simulink model "PID_SCHEME"  (R2024b)
settings: Solver=VariableStepAuto  StartTime=0.0  StopTime=10.0  RelTol=1e-3
undefined symbols (not defined in the file): a, b
libraries: slpidlib x1, px4Sensorslib x1, px4Peripheralslib x1
settings Model: Creator=xippa  LastModifiedBy=xippa

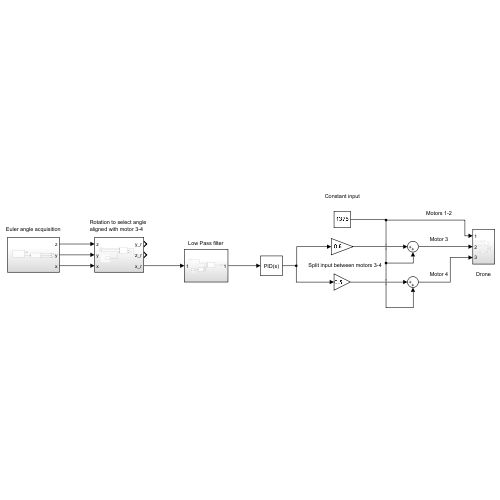
[thumbnail: Simulink's stored preview of the top-level diagram]
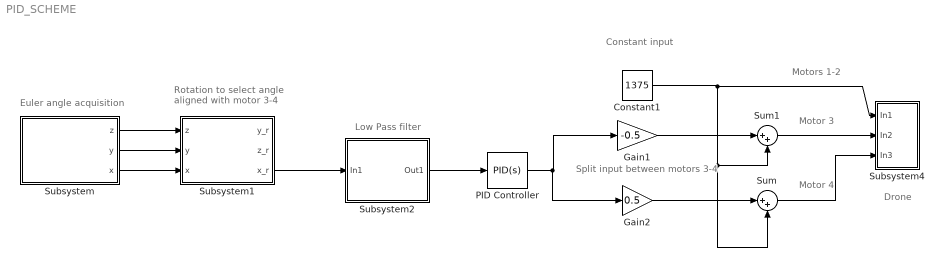
== system PID_SCHEME ==
  note: Drone
  note: Motor 4
  note: Motor 3
  note: Motors 1-2
  note: Constant input
  note: Split input between motors 3-4
  note: Low Pass filter
  note: Rotation to select angle
      | aligned with motor 3-4
  note: Euler angle acquisition
  Constant1 : Constant  Value=1375  SampleTime=0.001
  Gain1 : Gain  Gain=-0.5
  Gain2 : Gain  Gain=0.5
  PID Controller : slpidlib/PID Controller  Controller=PID  Form=Parallel  TimeDomain=Continuous-time  UseExternalTs=off  SampleTime=-1  IntegratorMethod=Forward Euler  FilterMethod=Forward Euler  ControllerParametersSource=internal  P=450  I=250  UseKiTs=off  D=100  UseExternalDerivativeSource=off  N=100  UseFilter=on  TunerSelectOption=Transfer Function Based (PID Tuner App)  InitialConditionSource=internal  InitialConditionForIntegrator=0  InitialConditionForFilter=0  DifferentiatorICPrevScaledInput=0  ExternalReset=none  TrackingMode=off  Kt=1  LimitOutput=off  SatLimitsSource=internal  UpperSaturationLimit=inf  LowerSaturationLimit=-inf  LinearizeAsGain=on  AntiWindupMode=none  Kb=1  LimitIntegrator=off  UpperIntegratorSaturationLimit=inf  LowerIntegratorSaturationLimit=-inf  POutMin=[]  POutMax=[]  IOutMin=[]  IOutMax=[]  DOutMin=[]  DOutMax=[]  NOutMin=[]  NOutMax=[]  SumOutMin=[]  SumOutMax=[]  SaturationOutMin=[]  SaturationOutMax=[]  PParamMin=[]  PParamMax=[]  IParamMin=[]  IParamMax=[]  DParamMin=[]  DParamMax=[]  NParamMin=[]  NParamMax=[]  KbParamMin=[]  KbParamMax=[]  KtParamMin=[]  KtParamMax=[]  KbOutMin=[]  KbOutMax=[]  KtOutMin=[]  KtOutMax=[]  IntegratorOutMin=[]  IntegratorOutMax=[]  FilterOutMin=[]  FilterOutMax=[]  SumI1OutMin=[]  SumI1OutMax=[]  SumI2OutMin=[]  SumI2OutMax=[]  SumI3OutMin=[]  SumI3OutMax=[]  SumI4OutMin=[]  SumI4OutMax=[]  SumDOutMin=[]  SumDOutMax=[]  DifferentiatorOutMin=[]  DifferentiatorOutMax=[]  FilterDiffOutCoefMin=[]  FilterDiffOutCoefMax=[]  ReciprocalOutMin=[]  ReciprocalOutMax=[]  SumDenOutMin=[]  SumDenOutMax=[]  SumNumOutMin=[]  SumNumOutMax=[]  DivideOutMin=[]  DivideOutMax=[]  UdiffTsProdOutMin=[]  UdiffTsProdOutMax=[]  NTsProdOutMin=[]  NTsProdOutMax=[]  UintegralTsProdOutMin=[]  UintegralTsProdOutMax=[]  UngainTsProdOutMin=[]  UngainTsProdOutMax=[]  ClampingZeroOutDataTypeStr=Inherit: Inherit via back propagation  ClampingZeroOutMin=[]  ClampingZeroOutMax=[]  FilterDenConstantOutDataTypeStr=Inherit: Inherit via back propagation  FilterDenConstantOutMin=[]  FilterDenConstantOutMax=[]  PCopyOutDataTypeStr=Inherit: Inherit via back propagation  PCopyOutMin=[]  PCopyOutMax=[]  NCopyOutDataTypeStr=Inherit: Inherit via back propagation  NCopyOutMin=[]  NCopyOutMax=[]  IntegratorContinuousStateAttributes=''  IntegratorStateMustResolveToSignalObject=off  IntegratorRTWStateStorageClass=Auto  FilterContinuousStateAttributes=''  FilterStateMustResolveToSignalObject=off  FilterRTWStateStorageClass=Auto  ParallelPVariant=InternalParameters  IdealPVariant=Disabled  IVariant=InternalParameters  DVariant=InternalParameters  IntegratorVariant=Continuous  SatVariant=Disabled  AWVariant=Passthrough  PCopyVariant=Disabled  TRVariant=Disabled  FdbkBlocksVariant=Forward  IdealPFdbkVariant=Disabled  SatFdbkVariant=Disabled  DerivativeFilterVariant=ContFilter  NVariant=InternalParameters  NCopyVariant=Disabled  FilterICVariant=InternalICsFilter  IntegratorICVariant=InternalICs  ExternalResetVariant=Disabled  TRSumVariant=Passthrough  SumFdbkVariant=Disabled  SumVariant=Sum_PID  TsampFilterVariant=InternalTs  TsampNgainVariant=Passthrough  TsampIntegralVariant=Disabled_SignalSpec  ExternalSaturationOutDataTypeStr=Inherit: Same as second input  DerivativeSourceVariant=ErrorSignal  PreIntVariant=InternalPreInt
  Subsystem : Subsystem
  Subsystem1 : Subsystem
  Subsystem2 : Subsystem
  Subsystem4 : Subsystem
  Sum : Sum  Inputs=|++
  Sum1 : Sum  Inputs=|++
  wires:
  Gain2/1 -> Sum/1
  PID Controller/1 -> Gain1/1, Gain2/1
  Gain1/1 -> Sum1/1
  Constant1/1 -> Sum1/2, Sum/2, Subsystem4/1(In1)
  Subsystem/1(z) -> Subsystem1/1(z)
  Subsystem/2(y) -> Subsystem1/2(y)
  Subsystem/3(x) -> Subsystem1/3(x)
  Subsystem1/3(x_r) -> Subsystem2/1(In1)
  Subsystem2/1(Out1) -> PID Controller/1
  Sum1/1 -> Subsystem4/2(In2)
  Sum/1 -> Subsystem4/3(In3)

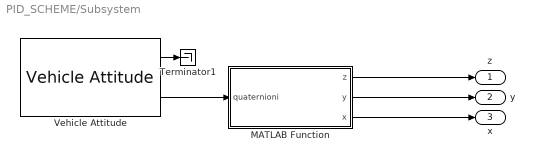
== system PID_SCHEME/Subsystem ==
  MATLAB Function : MATLAB Function  TreatAsAtomicUnit=on
  Terminator1 : Terminator
  Vehicle Attitude : px4Sensorslib/Vehicle Attitude  rollRate=off  pitchRate=off  yawRate=off  quaternion=on  uorbTimeStamp=off  BlockingMode=off  BlockTimeout=0.001  sampleTime=1/50
  z : Outport
  y : Outport  Port=2
  x : Outport  Port=3
  wires:
  Vehicle Attitude/2 -> MATLAB Function/1(quaternioni)
  Vehicle Attitude/1 -> Terminator1/1
  MATLAB Function/1(z) -> z/1
  MATLAB Function/3(x) -> x/1
  MATLAB Function/2(y) -> y/1

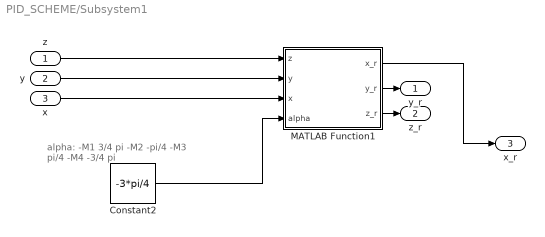
== system PID_SCHEME/Subsystem1 ==
  note: alpha:
      | -M1    3/4 pi
      | -M2    -pi/4
      | -M3    pi/4
      | -M4    -3/4 pi
  z : Inport
  y : Inport  Port=2
  x : Inport  Port=3
  Constant2 : Constant  Value=-3*pi/4
  MATLAB Function1 : MATLAB Function  TreatAsAtomicUnit=on
  y_r : Outport
  z_r : Outport  Port=2
  x_r : Outport  Port=3
  wires:
  x/1 -> MATLAB Function1/3(x)
  Constant2/1 -> MATLAB Function1/4(alpha)
  z/1 -> MATLAB Function1/1(z)
  MATLAB Function1/2(y_r) -> y_r/1
  MATLAB Function1/3(z_r) -> z_r/1
  y/1 -> MATLAB Function1/2(y)
  MATLAB Function1/1(x_r) -> x_r/1

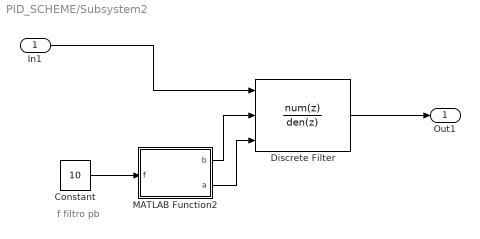
== system PID_SCHEME/Subsystem2 ==
  note: f filtro pb
  In1 : Inport
  Constant : Constant  Value=10
  Discrete Filter : DiscreteFilter  NumeratorSource=Input port  Numerator=b  DenominatorSource=Input port  Denominator=a  a0EqualsOne=on
      settings: InputPortMap=u0,p1,p3
  MATLAB Function2 : MATLAB Function  TreatAsAtomicUnit=on
  Out1 : Outport
  wires:
  In1/1 -> Discrete Filter/1
  MATLAB Function2/2(a) -> Discrete Filter/3
  MATLAB Function2/1(b) -> Discrete Filter/2
  Constant/1 -> MATLAB Function2/1(f)
  Discrete Filter/1 -> Out1/1

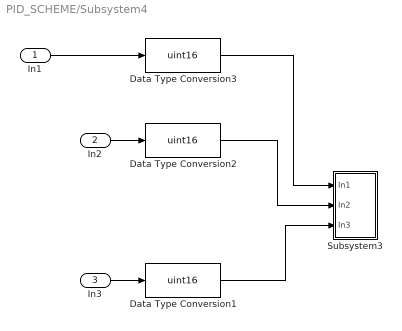
== system PID_SCHEME/Subsystem4 ==
  In1 : Inport
  In2 : Inport  Port=2
  In3 : Inport  Port=3
  Data Type Conversion1 : DataTypeConversion  OutDataTypeStr=uint16  SaturateOnIntegerOverflow=off  RndMeth=Floor
  Data Type Conversion2 : DataTypeConversion  OutDataTypeStr=uint16  SaturateOnIntegerOverflow=off  RndMeth=Floor
  Data Type Conversion3 : DataTypeConversion  OutDataTypeStr=uint16  SaturateOnIntegerOverflow=off  RndMeth=Floor
  Subsystem3 : Subsystem
  wires:
  In1/1 -> Data Type Conversion3/1
  Data Type Conversion1/1 -> Subsystem3/3(In3)
  Data Type Conversion3/1 -> Subsystem3/1(In1)
  Data Type Conversion2/1 -> Subsystem3/2(In2)
  In3/1 -> Data Type Conversion1/1
  In2/1 -> Data Type Conversion2/1

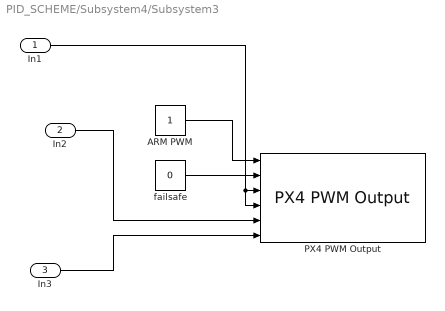
== system PID_SCHEME/Subsystem4/Subsystem3 ==
  In1 : Inport
  In2 : Inport  Port=2
  In3 : Inport  Port=3
  ARM PWM : Constant  OutDataTypeStr=boolean  SampleTime=0.001
  PX4 PWM Output : px4Peripheralslib/PX4 PWM Output  pwmDevice=Main  pwmChannel1_=on  pwmChannel2_=on  pwmChannel3_=on  pwmChannel4_=on  pwmChannel5_=off  pwmChannel6_=off  pwmChannel7_=off  pwmChannel8_=off
  failsafe : Constant  Value=0  OutDataTypeStr=boolean  SampleTime=0.001
  wires:
  ARM PWM/1 -> PX4 PWM Output/1
  failsafe/1 -> PX4 PWM Output/2
  In1/1 -> PX4 PWM Output/4, PX4 PWM Output/3
  In3/1 -> PX4 PWM Output/6
  In2/1 -> PX4 PWM Output/5

== matlab function PID_SCHEME/Subsystem1/MATLAB Function1 ==
  data: z input; y input; x input; x_r output; alpha input; y_r output; z_r output
function [x_r,y_r,z_r] = ruoto(z,y,x,alpha)
Global_POV = [x y z];
R_z = [cos(alpha), -sin(alpha), 0;
       sin(alpha), cos(alpha), 0;
       0, 0, 1];
LOCALPOV = Global_POV * R_z;
x_r = LOCALPOV(1);
y_r = LOCALPOV(2);
z_r = LOCALPOV(3);
end

== matlab function PID_SCHEME/Subsystem/MATLAB Function ==
  data: quaternioni input; z output; y output; x output
function [z, y, x] = fcn(quaternioni)
eulero = zeros(1,3);
eulero = quat2eul(quaternioni);
z = eulero(1);
y = eulero(2);
x = eulero(3);
end

== matlab function PID_SCHEME/Subsystem2/MATLAB Function2 ==
  data: f input; b output; a output
function [b,a] = BW(f)
fs = 1/50;
[b, a] = butter(1,f/(fs/2),'low');

end
